simulink model "dp7enc"  (R2026a)
settings: Solver=ode45  StopTime=15  RelTol=1e-6
InitFcn:
  | params7
values from neighbouring files (symbols this model uses):
  cpar = [kp kd ke dE tau_max Vin Vout]    [params.m]    (also in params7.m = [kE tau_sw tau_lqr Vin Vout kp_dn kd_dn])
  encpar = [dq_enc fc_vel Ts]    [params7.m]
  L1 = 0.5    [params.m]    (also in params7.m)
  L2 = 0.5    [params.m]    (also in params7.m = 0.4)
  p = [L1 W1 m1 L2 W2 m2 b1 b2 g]    [params.m]    (also in params7.m = [L1 lc1 m1 I1 L2 lc2 m2 I2 b1 b2 g])
  tau_sw = 3    [params7.m]
  W1 = 0.05    [params.m]    (also in params7.m = 0.03)
  W2 = 0.04    [params.m]    (also in params7.m = 0.03)
  x0 = [0.01; 0; 0; 0]    [params.m]    (also in params7.m)
undefined symbols (not defined in the file or in its folder): K, P
settings Model: SimulationMode=accelerator  Creator=ern  LastModifiedBy=ern

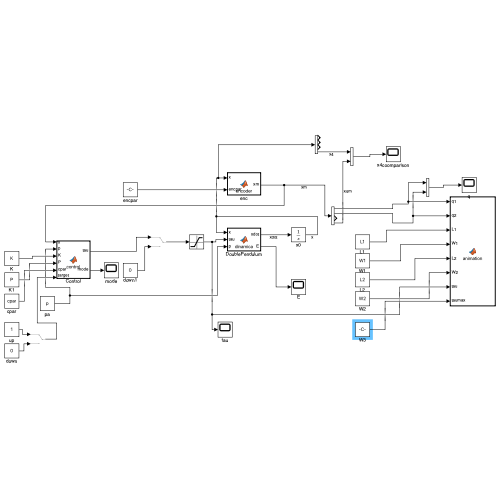
[thumbnail: Simulink's stored preview of the top-level diagram]
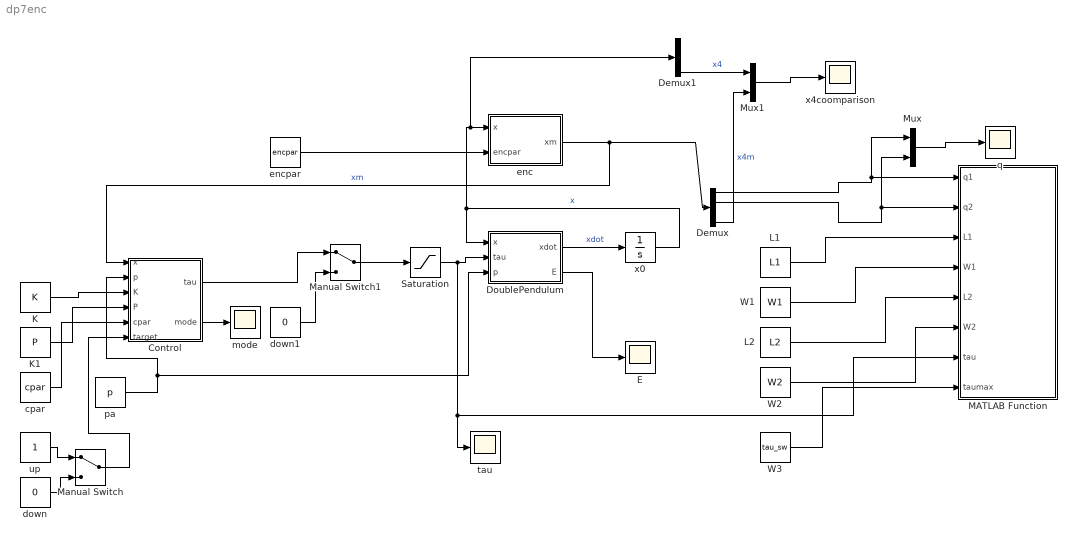
== system dp7enc ==
  Control : MATLAB Function  TreatAsAtomicUnit=on  SystemSampleTime=0.001
  Demux : Demux
  Demux1 : Demux
  DoublePendulum : MATLAB Function  TreatAsAtomicUnit=on
  E : Scope
      settings: ActiveDisplayYMinimum=-1  ActiveDisplayYMaximum=1
  K : Constant  Value=K
  K1 : Constant  Value=P  VectorParams1D=off
  L1 : Constant  Value=L1
  L2 : Constant  Value=L2
  MATLAB Function : MATLAB Function  TreatAsAtomicUnit=on  SystemSampleTime=0.01
  Manual Switch : ManualSwitch
  Manual Switch1 : ManualSwitch
  Mux : Mux  Inputs=2
  Mux1 : Mux  Inputs=2
  Saturation : Saturate  UpperLimit=tau_sw  LowerLimit=-tau_sw
  W1 : Constant  Value=W1
  W2 : Constant  Value=W2
  W3 : Constant  Value=tau_sw
  cpar : Constant  Value=cpar  VectorParams1D=off
  down : Constant  Value=0  VectorParams1D=off
  down1 : Constant  Value=0  VectorParams1D=off
  enc : MATLAB Function  TreatAsAtomicUnit=on  SystemSampleTime=0.001
  encpar : Constant  Value=encpar  VectorParams1D=off
  mode : Scope
      settings: ActiveDisplayYMinimum=-1  ActiveDisplayYMaximum=1  DataLoggingVariableName=ScopeData2
  pa : Constant  Value=p
  q : Scope
  tau : Scope
      settings: ActiveDisplayYMinimum=-1  ActiveDisplayYMaximum=1  DataLoggingVariableName=ScopeData3
  up : Constant  VectorParams1D=off
  x0 : Integrator  InitialCondition=x0
  x4coomparison : Scope
      settings: ActiveDisplayYMinimum=-0.096675800031018833  ActiveDisplayYMaximum=0.10598149201261475  DataLoggingVariableName=ScopeData4
  wires:
  L1/1 -> MATLAB Function/3(L1)
  W1/1 -> MATLAB Function/4(W1)
  L2/1 -> MATLAB Function/5(L2)
  W2/1 -> MATLAB Function/6(W2)
  pa/1 -> Control/2(p), DoublePendulum/3(p)
  DoublePendulum/1(xdot) -> x0/1  "xdot"
  x0/1 -> DoublePendulum/1(x), Demux1/1, enc/1(x)  "x"
  Demux/1 -> Mux/1, MATLAB Function/1(q1)
  Demux/2 -> Mux/2, MATLAB Function/2(q2)
  DoublePendulum/2(E) -> E/1
  Mux/1 -> q/1
  Control/1(tau) -> Manual Switch1/1
  K/1 -> Control/3(K)
  K1/1 -> Control/4(P)
  cpar/1 -> Control/5(cpar)
  Control/2(mode) -> mode/1
  up/1 -> Manual Switch/1
  down/1 -> Manual Switch/2
  Manual Switch/1 -> Control/6(target)
  encpar/1 -> enc/2(encpar)
  enc/1(xm) -> Control/1(x), Demux/1  "xm"
  Mux1/1 -> x4coomparison/1
  Demux1/4 -> Mux1/1  "x4"
  Demux/4 -> Mux1/2  "x4m"
  Saturation/1 -> MATLAB Function/7(tau), tau/1, DoublePendulum/2(tau)
  down1/1 -> Manual Switch1/2
  Manual Switch1/1 -> Saturation/1
  W3/1 -> MATLAB Function/8(taumax)

== matlab function dp7enc/DoublePendulum ==
  data: x input; xdot output; tau input; p input; E output
function [xdot, E] = dinamica(x, tau, p)
% Nonlinear dynamics of the double pendulum (q1 actuated, q2 passive)
%   M(q)*ddq + C(q,dq) + G(q) + F(dq) = [tau; 0]
% x   = [q1; q2; dq1; dq2]
%       q1: absolute angle of link 1 from the downward vertical (CCW positive)
%       q2: angle of link 2 relative to link 1
% tau = torque applied at joint 1 [N m]
% p   = [L1 lc1 m1 I1 L2 lc2 m2 I2 b1 b2 g]
% xdot = state derivative, E = total mechanical energy [J]

% --- Parameters
L1 = p(1); lc1 = p(2); m1 = p(3); I1 = p(4);   % link 1: length, CoM distance, mass, inertia about CoM
L2 = p(5); lc2 = p(6); m2 = p(7); I2 = p(8);   % link 2: length, CoM distance, mass, inertia about CoM
b1 = p(9); b2  = p(10); g = p(11);             % viscous friction coefficients, gravity

% --- State
q1 = x(1); q2 = x(2); dq1 = x(3); dq2 = x(4);
c2 = cos(q2); s2 = sin(q2);

% --- Inertia matrix (depends only on q2)
M11 = I1 + I2 + m1*lc1^2 + m2*(L1^2 + lc2^2 + 2*L1*lc2*c2);
M12 = I2 + m2*(lc2^2 + L1*lc2*c2);
M22 = I2 + m2*lc2^2;
M = [M11 M12; M12 M22];

% --- Coriolis and centrifugal terms
h = m2*L1*lc2*s2;
C = [-h*(2*dq1*dq2 + dq2^2); h*dq1^2];

% --- Gravity terms
G = [(m1*lc1 + m2*L1)*g*sin(q1) + m2*lc2*g*sin(q1+q2);
      m2*lc2*g*sin(q1+q2)];

% --- Viscous friction
F = [b1*dq1; b2*dq2];

% --- Joint accelerations (torque acts on joint 1 only)
dq  = [dq1; dq2];
ddq = M \ ([tau; 0] - C - G - F);
xdot = [dq; ddq];

% --- Total energy: kinetic + potential (V = 0 at the base joint, y pointing up)
E = 0.5*dq.'*M*dq - m1*g*lc1*cos(q1) - m2*g*(L1*cos(q1) + lc2*cos(q1+q2));
end

== matlab function dp7enc/MATLAB Function ==
  data: q1 input; q2 input; L1 input; W1 input; L2 input; W2 input; tau input; taumax input
function animation(q1, q2, L1, W1, L2, W2,tau,taumax)
coder.extrinsic('drawPendulum');
drawPendulum(q1, q2, L1, W1, L2, W2,tau,taumax);
end

== matlab function dp7enc/Control ==
  data: x input; tau output; p input; K input; P input; cpar input; mode output; target input
function [tau, mode] = control(x, p, K, P, cpar, target)
% Pure energy-pumping swing-up + LQR balancing
persistent m
if isempty(m), m = 0; end
L1 = p(1); lc1 = p(2); m1 = p(3); I1 = p(4);
L2 = p(5); lc2 = p(6); m2 = p(7); I2 = p(8); g = p(11);
kE = cpar(1); tau_sw = cpar(2); tau_lqr = cpar(3); Vin = cpar(4); Vout = cpar(5);
kp_dn = cpar(6); kd_dn = cpar(7);
q1 = x(1); q2 = x(2); dq1 = x(3); dq2 = x(4);
% Error with respect to the upright position
e = [atan2(sin(q1-pi), cos(q1-pi)); atan2(sin(q2), cos(q2)); dq1; dq2];
% Mode switching with hysteresis
V = e.'*P*e;
if target < 0.5
    m = 0;                          % down target: no LQR
elseif m == 0 && V < Vin
    m = 1;
elseif m == 1 && V > Vout
    m = 0;
end
if m == 1
    % --- LQR balancing ---
    tau = min(max(-K(:).'*e, -tau_lqr), tau_lqr);
else
    % --- Swing-up: energy pumping ---
    c2 = cos(q2);
    M11 = I1 + I2 + m1*lc1^2 + m2*(L1^2 + lc2^2 + 2*L1*lc2*c2);
    M12 = I2 + m2*(lc2^2 + L1*lc2*c2);
    M22 = I2 + m2*lc2^2;
    dq = [dq1; dq2];
    E    = 0.5*dq.'*[M11 M12; M12 M22]*dq ...
           - m1*g*lc1*cos(q1) - m2*g*(L1*cos(q1) + lc2*cos(q1+q2));
    Etop = (m1*lc1 + m2*(L1 + lc2))*g;
    if target > 0.5
        tau = min(max(kE*(Etop - E)*dq1, -tau_sw), tau_sw);       % pump energy up
    else
        e1dn = atan2(sin(q1), cos(q1));                            % error with respect to q1 = 0
        tau  = min(max(-kp_dn*e1dn - kd_dn*dq1, -tau_sw), tau_sw); % damped descent
    end
    %tau = min(max(kE*(Etop - E)*dq1, -tau_sw), tau_sw);
end
mode = m;
end

== matlab function dp7enc/enc ==
  data: x input; xm output; encpar input
function xm = encoder(x, encpar)
% Encoder quantizzati + stima velocità (differenza + passa-basso 1° ordine)
persistent qp vf
d1 = encpar(1); d2 = encpar(2); fc = encpar(3); Ts = encpar(4);

% Lettura encoder: quantizzazione (conteggio multigiro)
q = [round(x(1)/d1)*d1; round(x(2)/d2)*d2];

if isempty(qp)
    qp = q;  vf = [0; 0];
end

% Stima velocità
a  = exp(-2*pi*fc*Ts);
vr = (q - qp)/Ts;            % differenza finita
vf = a*vf + (1 - a)*vr;      % filtro passa-basso
qp = q;

xm = [q; vf];
end
